simulink model "Model_31_02_3"  (R2024b)
settings: Solver=FixedStepAuto  StartTime=0.0  StopTime=20  FixedStep=0.01  RelTol=1e-3
values from neighbouring files (symbols this model uses):
  b = pend1.b    [InversePODE.m]    (also in Laboratorio_2_Pendolo_inverso.m = 0.001; Laboratorio_2_Pendolo_inverso_conflict_copy_PC_2025_04_15.m = 13.516; Laboratorio_2_Pendolo_inverso_struct.m; TESTTT.m = 13.516)
  c = pend1.c    [InversePODE.m]    (also in Laboratorio_2_Pendolo_inverso.m = 0.1; Laboratorio_2_Pendolo_inverso_conflict_copy_PC_2025_04_15.m = 0.1; Laboratorio_2_Pendolo_inverso_struct.m; TESTTT.m = 0.1)
  F = -Kp*x_n_l_NL(:,3) - Kd * x_n_l_NL(:,4)    [Laboratorio_2_Pendolo_inverso.m]    (also in Laboratorio_2_Pendolo_inverso_conflict_copy_PC_2025_04_15.m; Laboratorio_2_Pendolo_inverso_struct.m; TESTTT.m)
  g = pend1.g    [InversePODE.m]    (also in Laboratorio_2_Pendolo_inverso.m = 9.81; Laboratorio_2_Pendolo_inverso_conflict_copy_PC_2025_04_15.m = 9.81; Laboratorio_2_Pendolo_inverso_struct.m; TESTTT.m = 9.81)
  l = pend1.l    [InversePODE.m]    (also in Laboratorio_2_Pendolo_inverso.m = 0.75; Laboratorio_2_Pendolo_inverso_conflict_copy_PC_2025_04_15.m = 0.75; Laboratorio_2_Pendolo_inverso_struct.m; TESTTT.m = 0.75)
  M = pend1.M    [InversePODE.m]    (also in Laboratorio_2_Pendolo_inverso.m = 3; Laboratorio_2_Pendolo_inverso_conflict_copy_PC_2025_04_15.m = 3; Laboratorio_2_Pendolo_inverso_struct.m; TESTTT.m = 3)
  m = pend1.m    [InversePODE.m]    (also in Laboratorio_2_Pendolo_inverso.m = 0.1; Laboratorio_2_Pendolo_inverso_conflict_copy_PC_2025_04_15.m = 0.1; Laboratorio_2_Pendolo_inverso_struct.m; TESTTT.m = 0.1)
settings Model: Creator=baron  LastModifiedBy=baron

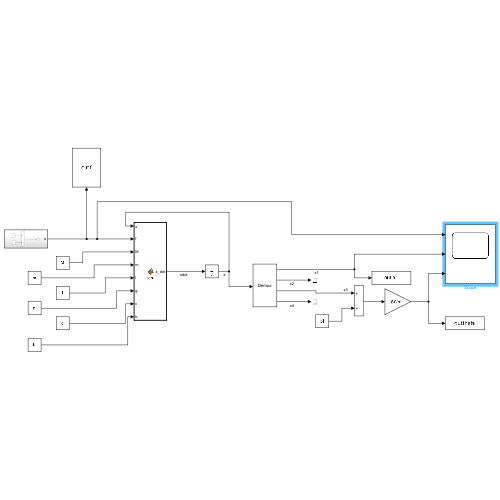
[thumbnail: Simulink's stored preview of the top-level diagram]
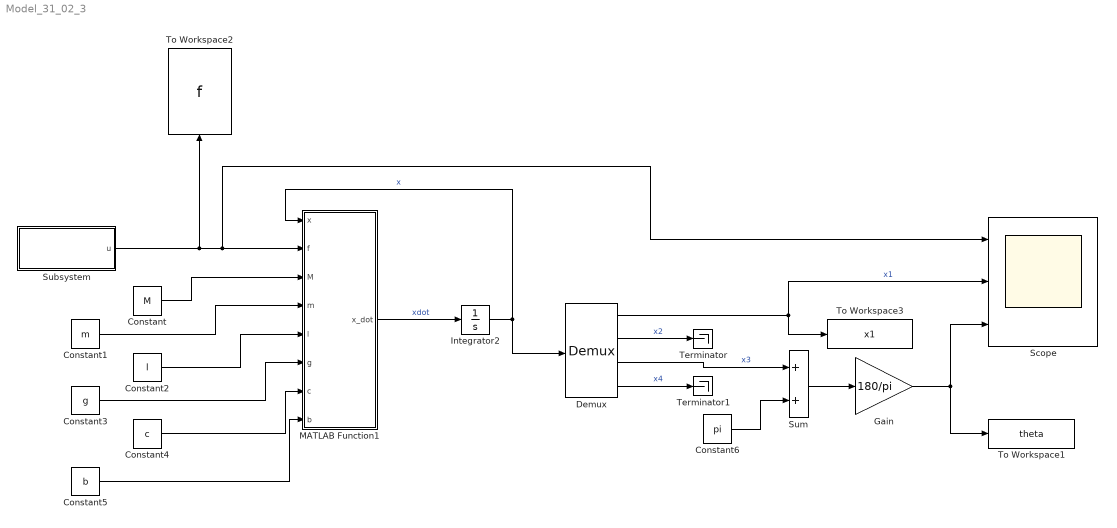
== system Model_31_02_3 ==
  Constant : Constant  Value=M
  Constant1 : Constant  Value=m
  Constant2 : Constant  Value=l
  Constant3 : Constant  Value=g
  Constant4 : Constant  Value=c
  Constant5 : Constant  Value=b
  Constant6 : Constant  Value=pi
  Demux : Demux
      settings: DisplayOption=none
  Gain : Gain  Gain=180/pi
  Integrator2 : Integrator  InitialCondition=[0;0;0;0]
  MATLAB Function1 : MATLAB Function  TreatAsAtomicUnit=on
  Scope : Scope  NumInputPorts=3
  Subsystem : Subsystem
  Sum : Sum
  Terminator : Terminator
  Terminator1 : Terminator
  To Workspace1 : ToWorkspace  VariableName=theta  SampleTime=-1
      settings: Save2DSignal=2-D array (concatenate along first dimension)
  To Workspace2 : ToWorkspace  VariableName=f  SampleTime=-1
      settings: Save2DSignal=2-D array (concatenate along first dimension)
  To Workspace3 : ToWorkspace  VariableName=x1  SampleTime=-1
      settings: Save2DSignal=2-D array (concatenate along first dimension)
  wires:
  Constant3/1 -> MATLAB Function1/6(g)
  Constant5/1 -> MATLAB Function1/8(b)
  Integrator2/1 -> Demux/1, MATLAB Function1/1(x)  "x"
  Constant/1 -> MATLAB Function1/3(M)
  MATLAB Function1/1(x_dot) -> Integrator2/1  "xdot"
  Demux/3 -> Sum/1  "x3"
  Gain/1 -> To Workspace1/1, Scope/3
  Constant2/1 -> MATLAB Function1/5(l)
  Demux/2 -> Terminator/1  "x2"
  Constant1/1 -> MATLAB Function1/4(m)
  Constant4/1 -> MATLAB Function1/7(c)
  Demux/1 -> Scope/2, To Workspace3/1  "x1"
  Subsystem/1(u) -> Scope/1, MATLAB Function1/2(f), To Workspace2/1
  Demux/4 -> Terminator1/1  "x4"
  Sum/1 -> Gain/1
  Constant6/1 -> Sum/2

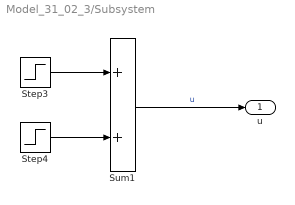
== system Model_31_02_3/Subsystem ==
  Step3 : Step  After=F  SampleTime=0
  Step4 : Step  Time=2  After=-F  SampleTime=0
  Sum1 : Sum
  u : Outport
  wires:
  Sum1/1 -> u/1  "u"
  Step4/1 -> Sum1/2
  Step3/1 -> Sum1/1

== matlab function Model_31_02_3/MATLAB Function1 ==
  data: x input; f input; x_dot output; M input; m input; l input; g input; c input; b input
function x_dot = fcn(x, f, M, m, l, g, c, b)
    
    A = [0 1 0 0; 0 -c/M (-m*g)/M -b/(M*l); 0 0 0 1; 0 -c/(M*l) (-g*(M+m))/(M*l) (-b*(M+m))/(M*m*(l^2))];
    B = [0; 1/M; 0; 1/(M*l)];

    x_dot = A * x + B * f;
    
end
